simulink model "day2"  (R2024a)
settings: Solver=VariableStepAuto  StartTime=0.0  StopTime=4  RelTol=1e-3
settings Model: Creator=user  LastModifiedBy=user

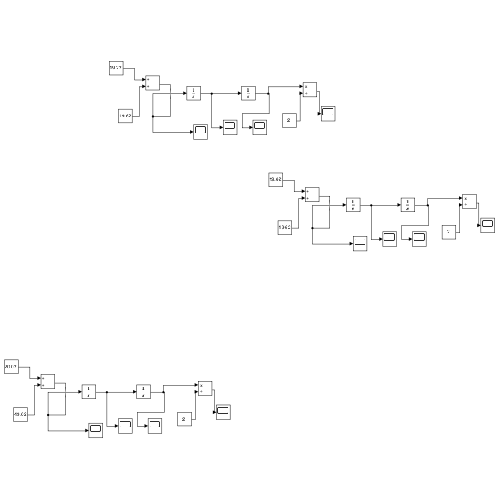
[thumbnail: Simulink's stored preview of the top-level diagram]
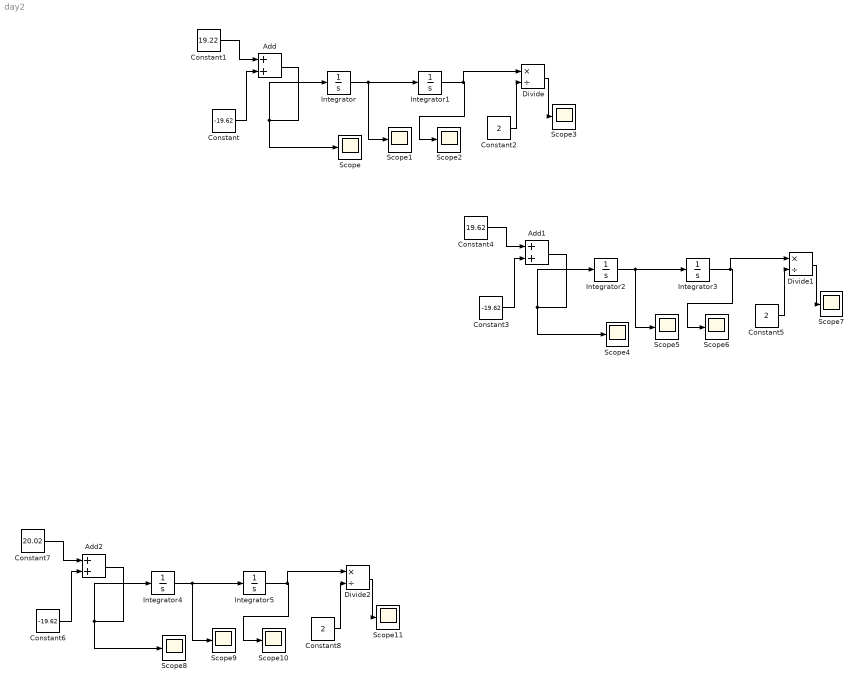
== system day2 ==
  Add : Sum
  Add1 : Sum
  Add2 : Sum
  Constant : Constant  Value=-19.62  SampleTime=0.002
  Constant1 : Constant  Value=19.22  SampleTime=0.02
  Constant2 : Constant  Value=2
  Constant3 : Constant  Value=-19.62  SampleTime=0.002
  Constant4 : Constant  Value=19.62  SampleTime=0.02
  Constant5 : Constant  Value=2
  Constant6 : Constant  Value=-19.62  SampleTime=0.002
  Constant7 : Constant  Value=20.02  SampleTime=0.02
  Constant8 : Constant  Value=2
  Divide : Product  Inputs=*/
  Divide1 : Product  Inputs=*/
  Divide2 : Product  Inputs=*/
  Integrator : Integrator  ContinuousStateAttributes="\"velocity\""
  Integrator1 : Integrator  ContinuousStateAttributes="\"altitude\""
  Integrator2 : Integrator  ContinuousStateAttributes="\"velocity\""
  Integrator3 : Integrator  ContinuousStateAttributes="\"altitude\""
  Integrator4 : Integrator  ContinuousStateAttributes="\"velocity\""
  Integrator5 : Integrator  ContinuousStateAttributes="\"altitude\""
  Scope{,1..11} (12 alike) : Scope
  wires:
  Add/1 -> Integrator/1, Scope/1
  Integrator/1 -> Scope1/1, Integrator1/1
  Integrator1/1 -> Divide/1, Scope2/1
  Constant1/1 -> Add/1
  Constant/1 -> Add/2
  Constant2/1 -> Divide/2
  Divide/1 -> Scope3/1
  Divide1/1 -> Scope7/1
  Add1/1 -> Integrator2/1, Scope4/1
  Constant4/1 -> Add1/1
  Integrator3/1 -> Divide1/1, Scope6/1
  Integrator2/1 -> Scope5/1, Integrator3/1
  Constant3/1 -> Add1/2
  Constant5/1 -> Divide1/2
  Divide2/1 -> Scope11/1
  Add2/1 -> Integrator4/1, Scope8/1
  Constant7/1 -> Add2/1
  Integrator5/1 -> Divide2/1, Scope10/1
  Integrator4/1 -> Scope9/1, Integrator5/1
  Constant6/1 -> Add2/2
  Constant8/1 -> Divide2/2
